simulink model "sf_yoyo"  (R2025b)
settings: Solver=ode23  StartTime=0.0  StopTime=500  FixedStep=1  RelTol=1e-3  EnableMultiTasking=on
settings Model: FPTRunName=Active  ExtModeTrigMode=oneshot  ExtModeArmWhenConnect=off  ExtModeAutoUpdateStatusClock=off  Creator=The MathWorks, Inc.  LastModifiedBy=The MathWorks, Inc.
settings SolverCC: AlgebraicLoopSolver=TrustRegion
settings DataIOCC: SaveFormat=Array  SaveOutput=off  SaveTime=off  ReturnWorkspaceOutputs=off
settings OptimizationCC: BlockReduction=off  BooleanDataType=off  OptimizeBlockIOStorage=off  BufferReuse=off  ReuseModelBlockBuffer=off  GlobalBufferReuse=off  ExpressionFolding=off  ExpressionDepthLimit=2147483647.0  LocalBlockOutputs=off  InitFltsAndDblsToZero=on  LifeSpan=inf  OptimizeDataStoreBuffers=off  BusAssignmentInplaceUpdate=off
settings DebuggingCC: SaveWithParameterizedLinksMsg=none  UnderspecifiedInitializationDetection=Classic  MergeDetectMultiDrivingBlocksExec=none  CheckExecutionContextPreStartOutputMsg=on  SignalResolutionControl=TryResolveAllWithWarning  MultiTaskDSMMsg=warning  MultiTaskCondExecSysMsg=none  FcnCallInpInsideContextMsg=warning  UnconnectedInputMsg=warning  UnconnectedOutputMsg=warning  UnconnectedLineMsg=warning  StateNameClashWarn=warning  SFUnexpectedBacktrackingDiag=warning  SFNoUnconditionalDefaultTransitionDiag=warning  SFExecutionAtInitializationDiag=none  ArithmeticOperatorsInVariantConditions=warning
settings HardwareCC: ProdBitPerPointer=32.0  ProdBitPerSizeT=32.0  ProdBitPerPtrDiffT=32.0  ProdLargestAtomicFloat=None  ProdIntDivRoundTo=Undefined  ProdEndianess=Unspecified  ProdWordSize=32.0  ProdHWDeviceType=32-bit Generic  TargetUnknown=on
settings ModelReferenceCC: EnableRefExpFcnMdlSchedulingChecks=on  PropagateSignalLabelsOutOfModel=off
settings SFSimCC: SimUseLocalCustomCode=off  SimParseCustomCode=off
settings RTWCC: RTWUseLocalCustomCode=off  GPUComputeCapability=3.5
settings CodeAppCC: StateflowObjectComments=on
settings GRTTargetCC: TargetFcnLib=ansi_tfl_tmw.mat  TargetLangStandard=C89/C90 (ANSI)  CombineOutputUpdateFcns=off  GRTInterface=on
settings ConfigComp: CovMetricSettings=dcmtr  CovSaveCumulativeToWorkspaceVar=on  CovSaveSingleToWorkspaceVar=on  CovExternalEMLEnable=off  CovSFcnEnable=off

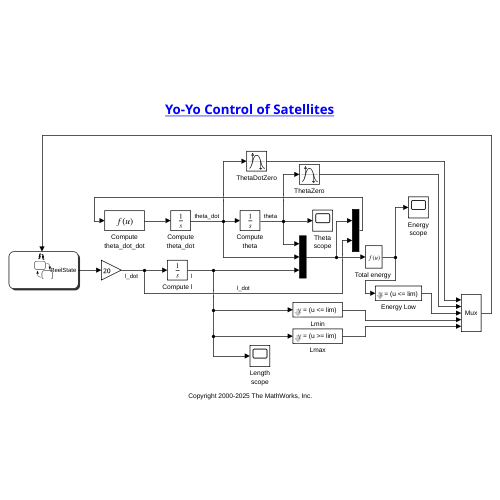
[thumbnail: Simulink's stored preview of the top-level diagram]
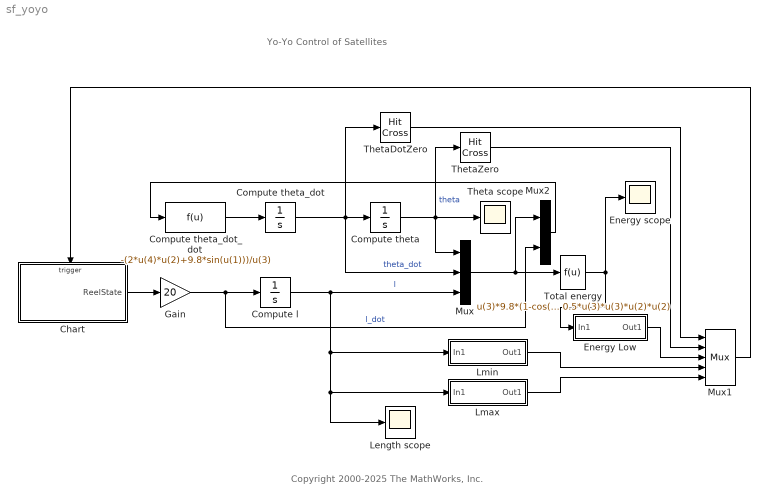
== system sf_yoyo ==
  note: Copyright 2000-2025 The MathWorks, Inc.
  note: Yo-Yo Control of Satellites
  Chart : Stateflow chart  TreatAsAtomicUnit=on
  Compute theta : Integrator  InitialCondition=0.16
  Compute theta_dot : Integrator
  Compute theta_dot_dot : Fcn  Expr=-(2*u(4)*u(2)+9.8*sin(u(1)))/u(3)
  Compute l : Integrator  InitialCondition=100  UpperSaturationLimit=105  LowerSaturationLimit=95
  Energy scope : Scope
      settings: TimeSpan=500  ActiveDisplayYMinimum=0  ActiveDisplayYMaximum=15  DataLoggingVariableName=EnergyTraj
  Energy Low : Subsystem  mask{th=0.001}
      mask prompts: th "Lower Limit"
      mask Display: disp('y = (u <= lim)')
  Gain : Gain  Gain=20  SaturateOnIntegerOverflow=on  OutDataTypeStr=Inherit: Same as input  ParamDataTypeStr=Inherit: Same as input
  Length scope : Scope
      settings: TimeSpan=500  ActiveDisplayYMinimum=90  ActiveDisplayYMaximum=110  DataLoggingVariableName=LengthTraj
  Lmax : Subsystem  mask{th=105}
      mask prompts: th "Upper Limit"
      mask Display: disp('y = (u >= lim)')
  Lmin : Subsystem  mask{th=95}
      mask prompts: th "Lower Limit"
      mask Display: disp('y = (u <= lim)')
  Mux : Mux  Inputs=3
  Mux1 : Mux  Inputs=5
  Mux2 : Mux  Inputs=2
  Theta scope : Scope
      settings: TimeSpan=500  ActiveDisplayYMinimum=-0.2  ActiveDisplayYMaximum=0.2  DataLoggingVariableName=ThetaTraj
  ThetaDotZero : HitCross
  ThetaZero : HitCross
  "Total energy " : Fcn  Expr=u(3)*9.8*(1-cos(u(1))) + 0.5*u(3)*u(3)*u(2)*u(2)
  wires:
  Compute theta_dot_dot/1 -> Compute theta_dot/1
  Chart/1(ReelState) -> Gain/1
  Compute theta_dot/1 -> Compute theta/1, ThetaDotZero/1, Mux/2  "theta_dot"
  Gain/1 -> Compute l/1, Mux2/2  "l_dot"
  Compute theta/1 -> ThetaZero/1, Theta scope/1, Mux/1  "theta"
  Mux1/1 -> Chart/Trigger
  Mux/1 -> "Total energy "/1, Mux2/1
  Energy Low/1(Out1) -> Mux1/3
  ThetaZero/1 -> Mux1/2
  ThetaDotZero/1 -> Mux1/1
  Compute l/1 -> Mux/3, Length scope/1, Lmax/1(In1), Lmin/1(In1)  "l"
  Mux2/1 -> Compute theta_dot_dot/1
  "Total energy "/1 -> Energy scope/1, Energy Low/1(In1)
  Lmin/1(Out1) -> Mux1/4
  Lmax/1(Out1) -> Mux1/5

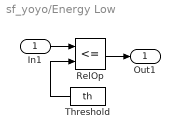
== system sf_yoyo/Energy Low ==
  In1 : Inport
  RelOp : RelationalOperator  Operator=<=  InputSameDT=off
  Threshold : Constant  Value=th
  Out1 : Outport  VectorParamsAs1DForOutWhenUnconnected=off
  wires:
  Threshold/1 -> RelOp/2
  In1/1 -> RelOp/1
  RelOp/1 -> Out1/1

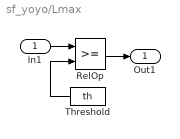
== system sf_yoyo/Lmax ==
  In1 : Inport
  RelOp : RelationalOperator  InputSameDT=off
  Threshold : Constant  Value=th
  Out1 : Outport  VectorParamsAs1DForOutWhenUnconnected=off
  wires:
  Threshold/1 -> RelOp/2
  In1/1 -> RelOp/1
  RelOp/1 -> Out1/1

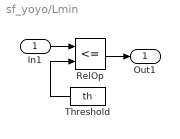
== system sf_yoyo/Lmin ==
  In1 : Inport
  RelOp : RelationalOperator  Operator=<=  InputSameDT=off
  Threshold : Constant  Value=th
  Out1 : Outport  VectorParamsAs1DForOutWhenUnconnected=off
  wires:
  RelOp/1 -> Out1/1
  In1/1 -> RelOp/1
  Threshold/1 -> RelOp/2

== stateflow chart sf_yoyo/Chart ==
  settings: sampleTime=1
  state Active
    state ReelMoving
      exit: ReelState = 0;
      state ReelOut
        entry: ReelState = 1;
      state ReelIn
        entry:ReelState= -1;
    state ReelStop
    (default) -> ReelStop
    ReelStop -> ReelOut [order 1] : ThetaZero
    ReelOut -> ReelStop : Lmax
    ReelIn -> ReelStop : Lmin
    ReelStop -> ReelIn [order 2] : ThetaDotZero
  state Inactive
  (default) -> Active : {ReelState = 0;}
  Active -> Inactive : EnergyLow
  data: ReelState output double size=1
  events: ThetaDotZero input EITHER_EDGE_EVENT; ThetaZero input EITHER_EDGE_EVENT; EnergyLow input EITHER_EDGE_EVENT; Lmin input EITHER_EDGE_EVENT; Lmax input EITHER_EDGE_EVENT
